simulink model "ilqar_lab4_2020b"  (R2020b)
settings: Solver=VariableStepAuto  StartTime=0.0  StopTime=10.0  RelTol=1e-3
libraries: dsparch4 x7
settings Model: Creator=Campus211  LastModifiedBy=Campus211

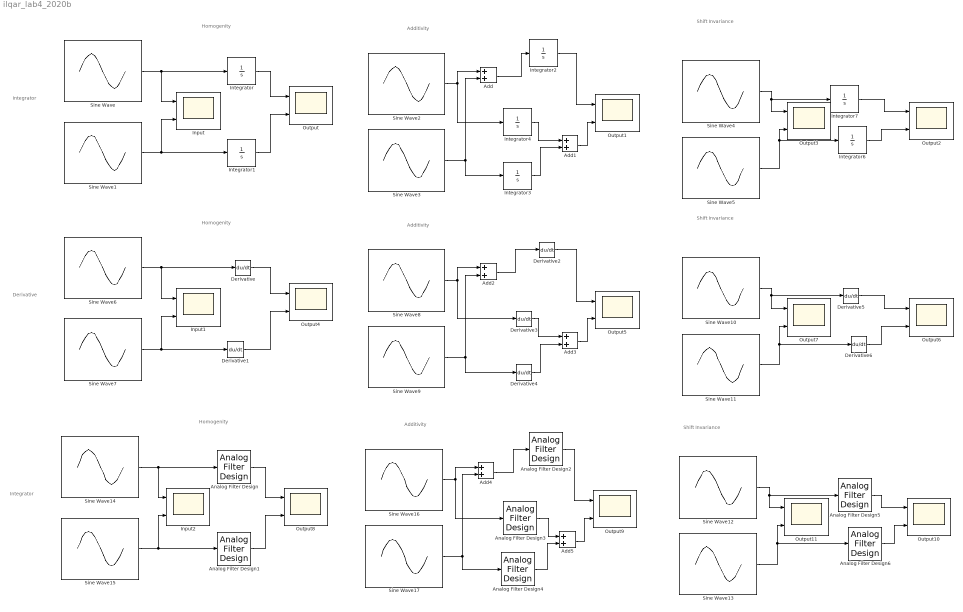
== system ilqar_lab4_2020b ==
  note: Integrator
  note: Homogenity
  note: Additivity
  note: Shift Invariance
  note: Shift Invariance
  note: Derivative
  note: Homogenity
  note: Additivity
  note: Homogenity
  note: Shift Invariance
  note: Integrator
  note: Additivity
  Add{,1..5} (6 alike) : Sum
  Analog Filter Design : dsparch4/Analog Filter Design  method=Butterworth  filttype=Lowpass  N=8  Wlo=0.5  Whi=80  Rp=2  Rs=40
  Analog Filter Design{1..6} (6 alike) : dsparch4/Analog Filter Design  method=Butterworth  filttype=Lowpass  N=8  Wlo=30  Whi=80  Rp=2  Rs=40
  Derivative{,1..6} (7 alike) : Derivative
  Input : Scope  NumInputPorts=2
  Input1 : Scope  NumInputPorts=2
  Input2 : Scope  NumInputPorts=2
  Integrator{,1..4,6..7} (7 alike) : Integrator
  Output{,1..11} (12 alike) : Scope  NumInputPorts=2
  Sine Wave{,5..6,11,13..14} (6 alike) : Sin  SampleTime=0
  Sine Wave1 : Sin  Amplitude=2  SampleTime=0
  Sine Wave10 : Sin  Phase=0.5*pi  SampleTime=0
  Sine Wave12 : Sin  Phase=0.5*pi  SampleTime=0
  Sine Wave15 : Sin  Amplitude=2  SampleTime=0
  Sine Wave16 : Sin  Amplitude=2  Frequency=5  SampleTime=0
  Sine Wave17 : Sin  Amplitude=5  Frequency=15  SampleTime=0
  Sine Wave2 : Sin  Amplitude=2  Frequency=5  SampleTime=0
  Sine Wave3 : Sin  Amplitude=5  Frequency=15  SampleTime=0
  Sine Wave4 : Sin  Phase=0.5*pi  SampleTime=0
  Sine Wave7 : Sin  Amplitude=2  SampleTime=0
  Sine Wave8 : Sin  Amplitude=2  Frequency=5  SampleTime=0
  Sine Wave9 : Sin  Amplitude=5  Frequency=15  SampleTime=0
  wires:
  Sine Wave/1 -> Input/1, Integrator/1
  Sine Wave1/1 -> Input/2, Integrator1/1
  Integrator/1 -> Output/1
  Integrator1/1 -> Output/2
  Integrator2/1 -> Output1/1
  Sine Wave3/1 -> Add/2, Integrator3/1
  Sine Wave2/1 -> Add/1, Integrator4/1
  Add/1 -> Integrator2/1
  Integrator4/1 -> Add1/1
  Integrator3/1 -> Add1/2
  Add1/1 -> Output1/2
  Sine Wave4/1 -> Output3/1, Integrator7/1
  Sine Wave5/1 -> Output3/2, Integrator6/1
  Integrator7/1 -> Output2/1
  Integrator6/1 -> Output2/2
  Derivative5/1 -> Output6/1
  Derivative/1 -> Output4/1
  Derivative1/1 -> Output4/2
  Sine Wave7/1 -> Derivative1/1, Input1/2
  Derivative4/1 -> Add3/2
  Sine Wave8/1 -> Derivative3/1, Add2/1
  Sine Wave9/1 -> Derivative4/1, Add2/2
  Sine Wave10/1 -> Derivative5/1, Output7/1
  Sine Wave6/1 -> Derivative/1, Input1/1
  Add3/1 -> Output5/2
  Derivative6/1 -> Output6/2
  Derivative3/1 -> Add3/1
  Add2/1 -> Derivative2/1
  Derivative2/1 -> Output5/1
  Sine Wave11/1 -> Output7/2, Derivative6/1
  Analog Filter Design6/1 -> Output10/2
  Analog Filter Design5/1 -> Output10/1
  Sine Wave13/1 -> Analog Filter Design6/1, Output11/2
  Analog Filter Design/1 -> Output8/1
  Analog Filter Design2/1 -> Output9/1
  Analog Filter Design1/1 -> Output8/2
  Analog Filter Design3/1 -> Add5/1
  Sine Wave12/1 -> Analog Filter Design5/1, Output11/1
  Sine Wave17/1 -> Analog Filter Design4/1, Add4/2
  Sine Wave16/1 -> Analog Filter Design3/1, Add4/1
  Analog Filter Design4/1 -> Add5/2
  Add5/1 -> Output9/2
  Add4/1 -> Analog Filter Design2/1
  Sine Wave14/1 -> Analog Filter Design/1, Input2/1
  Sine Wave15/1 -> Analog Filter Design1/1, Input2/2
